simulink model "monitoreo"  (R2023a)
settings: Solver=VariableStepAuto  StartTime=0.0  StopTime=inf  RelTol=1e-3
libraries: instrumentseriallib x3
settings Model: Creator=alcid  LastModifiedBy=alcid

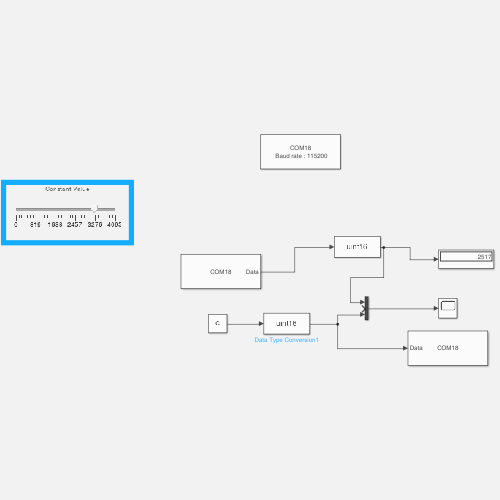
[thumbnail: Simulink's stored preview of the top-level diagram]
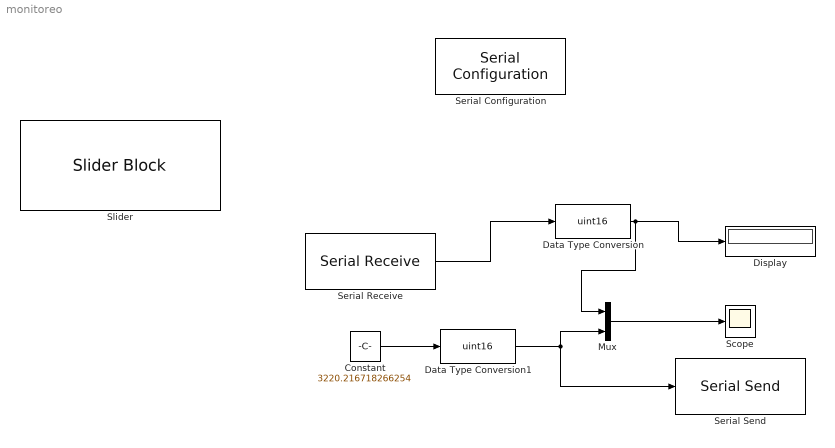
== system monitoreo ==
  Constant : Constant  Value=3220.216718266254
  Data Type Conversion : DataTypeConversion  OutDataTypeStr=uint16  SaturateOnIntegerOverflow=off  RndMeth=Floor
  Data Type Conversion1 : DataTypeConversion  OutDataTypeStr=uint16  SaturateOnIntegerOverflow=off  RndMeth=Floor
  Display : Display
  Mux : Mux  Inputs=3
  Scope : Scope
  Serial Configuration : instrumentseriallib/Serial Configuration  Priority=-200000  PortSel=COM18  Port=COM18  ComPort=COM18  BaudRate=115200  DataBits=8  Parity=none  StopBits=1  ByteOrder=little-endian  FlowControl=none  Timeout=10  SimulateUsing=Interpreted execution  BlockInModel=on  aMode=1
  Serial Receive : instrumentseriallib/Serial Receive  Priority=1  PortSel=COM18  Port=COM18  ComPort=COM18  DataType=uint16  SaveDataType=uint8  ToggleHeader=off  Header=[]  ToggleTerminator=off  Terminator=<none>  CustomTerminator=[]  InputFormat=Column major  ToggleDataSize=on  DataSize=[1 1]  EnableBlockingMode=on  ActionDataUnavailable=Output last received value  ActionWhenDataUnavailable=Output last received value  CustomValue=0  SampleTime=0.01  SimulateUsing=Interpreted execution  BlockInModel=on  aMode=1
  Serial Send : instrumentseriallib/Serial Send  Priority=1  PortSel=COM18  Port=COM18  ComPort=COM18  Header=[]  Terminator=<none>  CustomTerminator=[]  EnableBlockingMode=on  SimulateUsing=Interpreted execution  BlockInModel=on  aMode=1
  Slider : SliderBlock  ScaleMax=4095
  wires:
  Serial Receive/1 -> Data Type Conversion/1
  Data Type Conversion/1 -> Mux/1, Display/1
  Mux/1 -> Scope/1
  Constant/1 -> Data Type Conversion1/1
  Data Type Conversion1/1 -> Mux/3, Serial Send/1
